simulink library "BQ76952EVM"  (R2025b)
settings: Solver=VariableStepAuto  StartTime=0.0  StopTime=10.0  RelTol=1e-3
libraries: fl_lib x55, nesl_utility x20, ee_lib x2, simulink x1
settings Model: Creator=SC-Br  LastModifiedBy=SC-Br

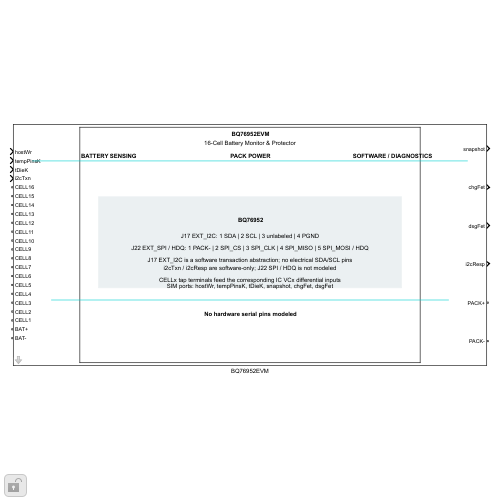
[thumbnail: Simulink's stored preview of the top-level diagram]
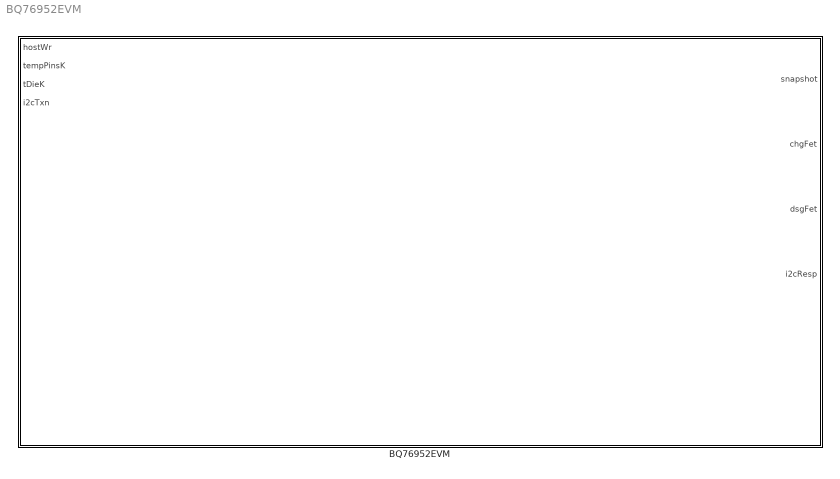
== system BQ76952EVM ==
  BQ76952EVM : Subsystem  mask(BQ76952EVM){SeriesCount=16, UsedCellMask=65535, CellSenseOhms=20, CellFilterFarads=220e-9, PositiveLinkOhms=1e-6, Preset=Generic 16S, ShuntOhms=0.001, DAConfig=6, SampleTime=0.01, PinConfig=[7 7 0 7 0 7 7 7 7], ProtEnabledA=188, ProtEnabledB=51, COV_Threshold=84, COV_Hyst=2, COV_Delay=74, CUV_Threshold=53, CUV_Hyst=2, CUV_Delay=74, OCC_Threshold=7, OCC_Delay=4, OCC_Recovery_mA=-200, OCD1_Threshold=28, OCD1_Delay=127, OCD_Recovery_mA=200, SCD_Threshold=5, SCD_Delay=2, SCD_Recovery_s=5, OTC_Threshold_C=45, OTC_Recovery_C=40, OTD_Threshold_C=60, OTD_Recovery_C=55, UTC_Threshold_C=0, UTC_Recovery_C=5, UTD_Threshold_C=-10, UTD_Recovery_C=-5, OTUT_Delay_s=2, RecoveryTime_s=3, MfgStatusInit=16, FetRon=0.001, FetGoff=1e-6, DisplayMode=Schematic View, I2CAddress=8}
      mask prompts: SeriesCount "Number of Series Cells"; UsedCellMask "Active VCell Mode (decimal)"; CellSenseOhms "VC series resistor (ohm)"; CellFilterFarads "VC filter capacitor (F)"; PositiveLinkOhms "BAT+ to PACK+ path resistance (ohm)"; Preset "Configuration preset"; ShuntOhms "Physical shunt resistance (ohm)"; DAConfig "DA_CONFIG data-memory byte"; SampleTime "Emulator sample time (s)"; PinConfig "Nine pin-configuration bytes"; ProtEnabledA "Protection enable A byte"; ProtEnabledB "Protection enable B byte"; COV_Threshold "COV threshold (50.6 mV units)"; COV_Hyst "COV recovery hysteresis (50.6 mV units)"; COV_Delay "COV delay (3.3 ms units)"; CUV_Threshold "CUV threshold (50.6 mV units)"; CUV_Hyst "CUV recovery hysteresis (50.6 mV units)"; CUV_Delay "CUV delay (3.3 ms units)"; OCC_Threshold "OCC threshold (2 mV per shunt)"; OCC_Delay "OCC delay code"; OCC_Recovery_mA "OCC recovery current (mA)"; OCD1_Threshold "OCD1 threshold (2 mV per shunt)"; OCD1_Delay "OCD1 delay code"; OCD_Recovery_mA "OCD recovery threshold (mA)"; SCD_Threshold "SCD threshold code"; SCD_Delay "SCD delay code"; SCD_Recovery_s "SCD recovery time (s)"; OTC_Threshold_C "OTC threshold (degC)"; OTC_Recovery_C "OTC recovery (degC)"; OTD_Threshold_C "OTD threshold (degC)"; OTD_Recovery_C "OTD recovery (degC)"; UTC_Threshold_C "UTC threshold (degC)"; UTC_Recovery_C "UTC recovery (degC)"; UTD_Threshold_C "UTD threshold (degC)"; UTD_Recovery_C "UTD recovery (degC)"; OTUT_Delay_s "OT/UT delay (s)"; RecoveryTime_s "Recovery time (s)"; MfgStatusInit "Manufacturing status initial word"; FetRon "Physical switch on resistance (ohm)"; FetGoff "Physical switch off conductance (S)"; DisplayMode "Display Mode"; I2CAddress "J17 I2C 7-bit address"
      mask help: Standalone behavioral BQ76952EVM. Conserving terminals retain fixed VC0-VC16 identities; use explicit external shorts for unused taps. J17 is available only through the transaction-level software interface.
      mask TypeOptions SeriesCount: 3 | 4 | 5 | 6 | 7 | 8 | 9 | 10 | 11 | 12 | 13 | 14 | 15 | 16
      mask Callback SeriesCount: n=str2double(get_param(gcb,'SeriesCount')); v=uint16(2^(n-1)-1+32768); if n==16, v=65535; end; set_param(gcb,'UsedCellMask',num2str(double(v)))
      mask TypeOptions Preset: Generic 16S | Solaris 13S | Generic 4S
      mask Callback Preset: switch get_param(gcb,'Preset'), case 'Solaris 13S', set_param(gcb,'SeriesCount','13'); set_param(gcb,'UsedCellMask','36863'); set_param(gcb,'DAConfig','6'); set_param(gcb,'ShuntOhms','0.001'); case 'Generic 4S', set_param(gcb,'SeriesCount','4'); set_param(gcb,'UsedCellMask','32775'); case 'Generic 16S', set_param(gcb,'SeriesCount','16'); set_param(gcb,'UsedCellMask','65535'); end
      mask TypeOptions DisplayMode: PCB View | Schematic View
      mask DialogControl BatteryCells Prompt: Battery / cell configuration
      mask DialogControl Current Prompt: Current sensing
      mask DialogControl Acquisition Prompt: Voltage and temperature acquisition
      mask DialogControl Protection Prompt: Protection thresholds and recovery
      mask DialogControl FETs Prompt: FET behaviour
      mask DialogControl Communications Prompt: Communications and diagnostics
      mask DialogControl ProtocolNote Prompt: J17 software transaction interface: i2cTxn (40-byte request) / i2cResp (40-byte response); supports device address, ACK/NACK, direct registers, data memory and implemented subcommands. This is not an electrical SDA/SCL waveform model. J22 SPI/HDQ is not implemented as a functional interface.
      mask Display: if DisplayMode == 1, color('white'); patch([0 1 1 0],[0 0 1 1],[1 1 1]); image(imread(fullfile(fileparts(which('BQ76952EVM')),'assets','bq76952evm_top_cropped.png')),[0.18 0.0125 0.64 0.975]); port_label('lconn',1,'CELL16'); port_label('lconn',2,'CELL15'); port_label('lconn',3,'CELL14'); port_label('lconn',4,'CELL13'); port_label('lconn',5,'CELL12'); port_label('lconn',6,'CELL11'); port_label('lconn',7,'CELL10'); port_label('lconn',8,'CELL9'); port_label('lconn',9,'CELL8'); port_label('lconn',10,'CELL7'); port_label('lconn',11,'CELL6'); port_label('lconn',12,'CELL5'); port_label('lconn',13,'CELL4'); port_label('lconn',14,'CELL3'); port_label('lconn',15,'CELL2'); port_label('lconn',16,'CELL1'); port_label('lconn',17,'BAT+'); port_label('lconn',18,'BAT-'); port_label('rconn',1,'PACK+'); port_label('rconn',2,'PACK-'); port_label('input',1,'SIM hostWr'); port_label('input',2,'SIM tempPinsK'); port_label('input',3,'SIM tDieK'); port_label('input',4,'I2C transaction request (SW)'); port_label('output',1,'SIM snapshot'); port_label('output',2,'SIM chgFet status'); port_label('output',3,'SIM dsgFet status'); port_label('output',4,'I2C transaction response (SW)'); else, color('white'); patch([0.14 0.86 0.86 0.14],[0.01 0.01 0.99 0.99],[1 1 1]); color('black'); plot([0.14 0.86 0.86 0.14 0.14],[0.01 0.01 0.99 0.99 0.01]); text(0.5,0.965,'{\bf BQ76952EVM}','horizontalAlignment','center','texmode','on'); text(0.5,0.925,'16-Cell Battery Monitor & Protector','horizontalAlignment','center'); color('black'); text(0.20,0.875,'{\bf BATTERY SENSING}','horizontalAlignment','center','texmode','on'); text(0.50,0.875,'{\bf PACK POWER}','horizontalAlignment','center','texmode','on'); text(0.80,0.875,'{\bf SOFTWARE / DIAGNOSTICS}','horizontalAlignment','center','texmode','on'); color('cyan'); plot([0.04 0.96],[0.85 0.85]); color('white'); patch([0.18 0.82 0.82 0.18],[0.32 0.32 0.70 0.70],[0.92 0.94 0.95]); color('black'); text(0.5,0.61,'{\bf BQ76952}','horizontalAlignment','center','texmode','on'); text(0.5,0.54,'J17 EXT_I2C: 1 SDA | 2 SCL | 3 unlabeled | 4 PGND','horizontalAlignment','center'); text(0.5,0.49,'J22 EXT_SPI / HDQ: 1 PACK- | 2 SPI_CS | 3 SPI_CLK | 4 SPI_MISO | 5 SPI_MOSI / HDQ','horizontalAlignment','center'); text(0.5,0.44,'J17 EXT_I2C is a software transaction abstraction; no electrical SDA/SCL pins','horizontalAlignment','center'); text(0.5,0.405,'i2cTxn / i2cResp are software-only; J22 SPI / HDQ is not modeled','horizontalAlignment','center'); text(0.5,0.355,'CELLx tap terminals feed the corresponding IC VCx differential inputs','horizontalAlignment','center'); text(0.5,0.33,'SIM ports: hostWr, tempPinsK, tDieK, snapshot, chgFet, dsgFet','horizontalAlignment','center'); color('cyan'); plot([0.08 0.92],[0.27 0.27]); color('black'); text(0.5,0.22,'{\bf No hardware serial pins modeled}','horizontalAlignment','center','texmode','on'); end

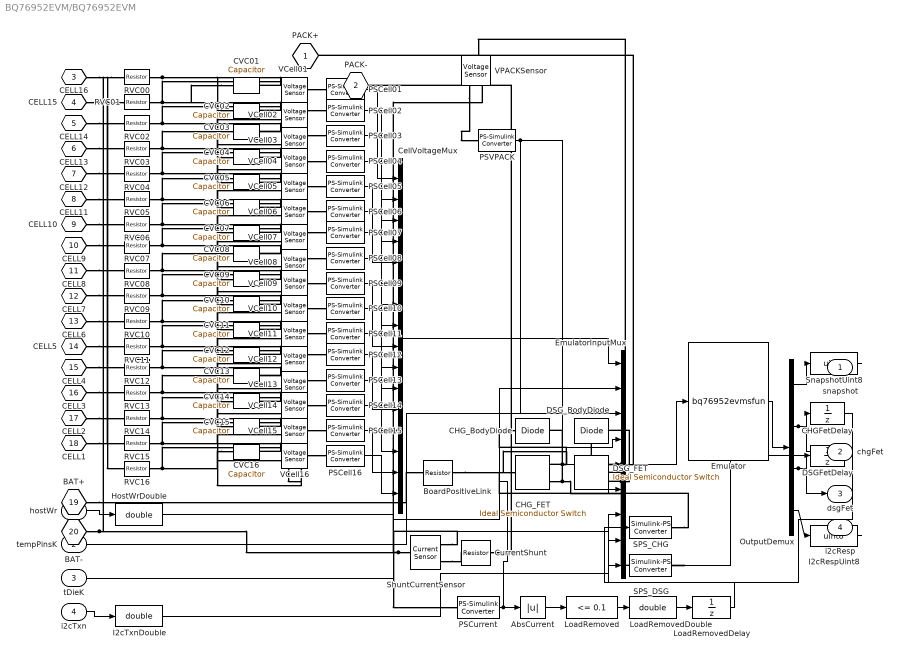
== system BQ76952EVM/BQ76952EVM ==
  hostWr : Inport  OutDataTypeStr=uint8  PortDimensions=40
  tempPinsK : Inport  Port=2  OutDataTypeStr=double  PortDimensions=9
  tDieK : Inport  Port=3  OutDataTypeStr=double  PortDimensions=1
  i2cTxn : Inport  Port=4  OutDataTypeStr=uint8  PortDimensions=40
  AbsCurrent : Abs  SaturateOnIntegerOverflow=off
  BoardPositiveLink : fl_lib/Electrical/Electrical Elements/Resistor  R=PositiveLinkOhms Ohm  i_specify=off  i_priority=None  i=0 A  i_nominal_specify=off  i_nominal_value=1  i_nominal_unit=A  v_specify=off  v_priority=None  v=0 V  v_nominal_specify=off  v_nominal_value=1  v_nominal_unit=V
  CHGFetDelay : UnitDelay  InitialCondition=1  SampleTime=SampleTime  HasFrameUpgradeWarning=on
  CHG_BodyDiode : fl_lib/Electrical/Electrical Elements/Diode  Vf=0.7 V  Ron=0.01 Ohm  Goff=FetGoff 1/Ohm  i_specify=off  i_priority=None  i=0 A  i_nominal_specify=off  i_nominal_value=1  i_nominal_unit=A  v_specify=off  v_priority=None  v=0 V  v_nominal_specify=off  v_nominal_value=1  v_nominal_unit=V
  CHG_FET : ee_lib/Semiconductors & Converters/Ideal Semiconductor Switch  port_option=ee.enum.controlport.ps  Ron=FetRon Ohm  Goff=FetGoff 1/Ohm  Vth=0.5 V  diode_param=ee.enum.semiconductors.protectionDiode.external  diode_Vf=0.8 V  diode_Ron=0.001 Ohm  diode_Goff=1e-5 1/Ohm  diode_C=50e-9 F  diode_iRM=-235 A  diode_iF=300 A  diode_idot=-50 A/us  diode_trr_param=ee.enum.converters.diodetrr.trr_factor  diode_trr_factor=3  diode_trr=15 us  diode_Qrr=1500 s*uA
  CVC01 : fl_lib/Electrical/Electrical Elements/Capacitor  c=CellFilterFarads F  r=1e-6 Ohm  g=0 1/Ohm  i_specify=off  i_priority=None  i=0 A  i_nominal_specify=off  i_nominal_value=1  i_nominal_unit=A  v_specify=off  v_priority=None  v=0 V  v_nominal_specify=off  v_nominal_value=1  v_nominal_unit=V  vc_specify=off  vc_priority=High  vc=0 V  vc_nominal_specify=off  vc_nominal_value=1  vc_nominal_unit=V
  CVC02 : fl_lib/Electrical/Electrical Elements/Capacitor  c=CellFilterFarads F  r=1e-6 Ohm  g=0 1/Ohm  i_specify=off  i_priority=None  i=0 A  i_nominal_specify=off  i_nominal_value=1  i_nominal_unit=A  v_specify=off  v_priority=None  v=0 V  v_nominal_specify=off  v_nominal_value=1  v_nominal_unit=V  vc_specify=off  vc_priority=High  vc=0 V  vc_nominal_specify=off  vc_nominal_value=1  vc_nominal_unit=V
  CVC03 : fl_lib/Electrical/Electrical Elements/Capacitor  c=CellFilterFarads F  r=1e-6 Ohm  g=0 1/Ohm  i_specify=off  i_priority=None  i=0 A  i_nominal_specify=off  i_nominal_value=1  i_nominal_unit=A  v_specify=off  v_priority=None  v=0 V  v_nominal_specify=off  v_nominal_value=1  v_nominal_unit=V  vc_specify=off  vc_priority=High  vc=0 V  vc_nominal_specify=off  vc_nominal_value=1  vc_nominal_unit=V
  CVC04 : fl_lib/Electrical/Electrical Elements/Capacitor  c=CellFilterFarads F  r=1e-6 Ohm  g=0 1/Ohm  i_specify=off  i_priority=None  i=0 A  i_nominal_specify=off  i_nominal_value=1  i_nominal_unit=A  v_specify=off  v_priority=None  v=0 V  v_nominal_specify=off  v_nominal_value=1  v_nominal_unit=V  vc_specify=off  vc_priority=High  vc=0 V  vc_nominal_specify=off  vc_nominal_value=1  vc_nominal_unit=V
  CVC05 : fl_lib/Electrical/Electrical Elements/Capacitor  c=CellFilterFarads F  r=1e-6 Ohm  g=0 1/Ohm  i_specify=off  i_priority=None  i=0 A  i_nominal_specify=off  i_nominal_value=1  i_nominal_unit=A  v_specify=off  v_priority=None  v=0 V  v_nominal_specify=off  v_nominal_value=1  v_nominal_unit=V  vc_specify=off  vc_priority=High  vc=0 V  vc_nominal_specify=off  vc_nominal_value=1  vc_nominal_unit=V
  CVC06 : fl_lib/Electrical/Electrical Elements/Capacitor  c=CellFilterFarads F  r=1e-6 Ohm  g=0 1/Ohm  i_specify=off  i_priority=None  i=0 A  i_nominal_specify=off  i_nominal_value=1  i_nominal_unit=A  v_specify=off  v_priority=None  v=0 V  v_nominal_specify=off  v_nominal_value=1  v_nominal_unit=V  vc_specify=off  vc_priority=High  vc=0 V  vc_nominal_specify=off  vc_nominal_value=1  vc_nominal_unit=V
  CVC07 : fl_lib/Electrical/Electrical Elements/Capacitor  c=CellFilterFarads F  r=1e-6 Ohm  g=0 1/Ohm  i_specify=off  i_priority=None  i=0 A  i_nominal_specify=off  i_nominal_value=1  i_nominal_unit=A  v_specify=off  v_priority=None  v=0 V  v_nominal_specify=off  v_nominal_value=1  v_nominal_unit=V  vc_specify=off  vc_priority=High  vc=0 V  vc_nominal_specify=off  vc_nominal_value=1  vc_nominal_unit=V
  CVC08 : fl_lib/Electrical/Electrical Elements/Capacitor  c=CellFilterFarads F  r=1e-6 Ohm  g=0 1/Ohm  i_specify=off  i_priority=None  i=0 A  i_nominal_specify=off  i_nominal_value=1  i_nominal_unit=A  v_specify=off  v_priority=None  v=0 V  v_nominal_specify=off  v_nominal_value=1  v_nominal_unit=V  vc_specify=off  vc_priority=High  vc=0 V  vc_nominal_specify=off  vc_nominal_value=1  vc_nominal_unit=V
  CVC09 : fl_lib/Electrical/Electrical Elements/Capacitor  c=CellFilterFarads F  r=1e-6 Ohm  g=0 1/Ohm  i_specify=off  i_priority=None  i=0 A  i_nominal_specify=off  i_nominal_value=1  i_nominal_unit=A  v_specify=off  v_priority=None  v=0 V  v_nominal_specify=off  v_nominal_value=1  v_nominal_unit=V  vc_specify=off  vc_priority=High  vc=0 V  vc_nominal_specify=off  vc_nominal_value=1  vc_nominal_unit=V
  CVC{10..16} (7 alike) : fl_lib/Electrical/Electrical Elements/Capacitor  c=CellFilterFarads F  r=1e-6 Ohm  g=0 1/Ohm  i_specify=off  i_priority=None  i=0 A  i_nominal_specify=off  i_nominal_value=1  i_nominal_unit=A  v_specify=off  v_priority=None  v=0 V  v_nominal_specify=off  v_nominal_value=1  v_nominal_unit=V  vc_specify=off  vc_priority=High  vc=0 V  vc_nominal_specify=off  vc_nominal_value=1  vc_nominal_unit=V
  CellVoltageMux : Mux  Inputs=16
  CurrentShunt : fl_lib/Electrical/Electrical Elements/Resistor  R=ShuntOhms Ohm  i_specify=off  i_priority=None  i=0 A  i_nominal_specify=off  i_nominal_value=1  i_nominal_unit=A  v_specify=off  v_priority=None  v=0 V  v_nominal_specify=off  v_nominal_value=1  v_nominal_unit=V
  DSGFetDelay : UnitDelay  InitialCondition=1  SampleTime=SampleTime  HasFrameUpgradeWarning=on
  DSG_BodyDiode : fl_lib/Electrical/Electrical Elements/Diode  Vf=0.7 V  Ron=0.01 Ohm  Goff=FetGoff 1/Ohm  i_specify=off  i_priority=None  i=0 A  i_nominal_specify=off  i_nominal_value=1  i_nominal_unit=A  v_specify=off  v_priority=None  v=0 V  v_nominal_specify=off  v_nominal_value=1  v_nominal_unit=V
  DSG_FET : ee_lib/Semiconductors & Converters/Ideal Semiconductor Switch  port_option=ee.enum.controlport.ps  Ron=FetRon Ohm  Goff=FetGoff 1/Ohm  Vth=0.5 V  diode_param=ee.enum.semiconductors.protectionDiode.external  diode_Vf=0.8 V  diode_Ron=0.001 Ohm  diode_Goff=1e-5 1/Ohm  diode_C=50e-9 F  diode_iRM=-235 A  diode_iF=300 A  diode_idot=-50 A/us  diode_trr_param=ee.enum.converters.diodetrr.trr_factor  diode_trr_factor=3  diode_trr=15 us  diode_Qrr=1500 s*uA
  Emulator : S-Function  FunctionName=bq76952evmsfun  Parameters=[SampleTime; UsedCellMask; round(ShuntOhms*1e6); DAConfig; ProtEnabledA; ProtEnabledB; MfgStatusInit; COV_Threshold; COV_Hyst; COV_Delay; CUV_Threshold; CUV_Hyst; CUV_Delay; OCC_Threshold; OCC_Delay; OCC_Recovery_mA; OCD1_Threshold; OCD1_Delay; OCD_Recovery_mA; SCD_Threshold; SCD_Delay; SCD_Recovery_s; OTC_Threshold_C; OTC_Recovery_C; OTD_Threshold_C; OTD_Recovery_C; UTC_Threshold_C; UTC_Recovery_C; UTD_Threshold_C; UTD_Recovery_C; OTUT_Delay_s; RecoveryTime_s; PinConfig(:); I2CAddress]  SFunctionDeploymentMode=off  EnableBusSupport=off
  EmulatorInputMux : Mux  Inputs=9
  HostWrDouble : DataTypeConversion  OutDataTypeStr=double  SaturateOnIntegerOverflow=off  RndMeth=Floor
  I2cRespUint8 : DataTypeConversion  OutDataTypeStr=uint8  SaturateOnIntegerOverflow=off  RndMeth=Floor
  I2cTxnDouble : DataTypeConversion  OutDataTypeStr=double  SaturateOnIntegerOverflow=off  RndMeth=Floor
  LoadRemoved : simulink/Logic and Bit Operations/Compare To Constant  relop=<=  const=0.1  OutDataTypeStr=boolean
  LoadRemovedDelay : UnitDelay  SampleTime=SampleTime  HasFrameUpgradeWarning=on
  LoadRemovedDouble : DataTypeConversion  OutDataTypeStr=double  SaturateOnIntegerOverflow=off  RndMeth=Floor
  OutputDemux : Demux  Outputs=[144 1 1 40]
  PSCell01 : nesl_utility/PS-Simulink Converter  PhysicalDomain=network_engine_domain  SubClassName=ps_output  LeftPortType=input  RightPortType=output  PseudoPeriodic=off  Frequencies=[]  VectorFormat=inherit  Unit=inherit  AffineConversion=off
  PSCell02 : nesl_utility/PS-Simulink Converter  PhysicalDomain=network_engine_domain  SubClassName=ps_output  LeftPortType=input  RightPortType=output  PseudoPeriodic=off  Frequencies=[]  VectorFormat=inherit  Unit=inherit  AffineConversion=off
  PSCell03 : nesl_utility/PS-Simulink Converter  PhysicalDomain=network_engine_domain  SubClassName=ps_output  LeftPortType=input  RightPortType=output  PseudoPeriodic=off  Frequencies=[]  VectorFormat=inherit  Unit=inherit  AffineConversion=off
  PSCell04 : nesl_utility/PS-Simulink Converter  PhysicalDomain=network_engine_domain  SubClassName=ps_output  LeftPortType=input  RightPortType=output  PseudoPeriodic=off  Frequencies=[]  VectorFormat=inherit  Unit=inherit  AffineConversion=off
  PSCell05 : nesl_utility/PS-Simulink Converter  PhysicalDomain=network_engine_domain  SubClassName=ps_output  LeftPortType=input  RightPortType=output  PseudoPeriodic=off  Frequencies=[]  VectorFormat=inherit  Unit=inherit  AffineConversion=off
  PSCell06 : nesl_utility/PS-Simulink Converter  PhysicalDomain=network_engine_domain  SubClassName=ps_output  LeftPortType=input  RightPortType=output  PseudoPeriodic=off  Frequencies=[]  VectorFormat=inherit  Unit=inherit  AffineConversion=off
  PSCell07 : nesl_utility/PS-Simulink Converter  PhysicalDomain=network_engine_domain  SubClassName=ps_output  LeftPortType=input  RightPortType=output  PseudoPeriodic=off  Frequencies=[]  VectorFormat=inherit  Unit=inherit  AffineConversion=off
  PSCell08 : nesl_utility/PS-Simulink Converter  PhysicalDomain=network_engine_domain  SubClassName=ps_output  LeftPortType=input  RightPortType=output  PseudoPeriodic=off  Frequencies=[]  VectorFormat=inherit  Unit=inherit  AffineConversion=off
  PSCell09 : nesl_utility/PS-Simulink Converter  PhysicalDomain=network_engine_domain  SubClassName=ps_output  LeftPortType=input  RightPortType=output  PseudoPeriodic=off  Frequencies=[]  VectorFormat=inherit  Unit=inherit  AffineConversion=off
  PSCell{10..16} (7 alike) : nesl_utility/PS-Simulink Converter  PhysicalDomain=network_engine_domain  SubClassName=ps_output  LeftPortType=input  RightPortType=output  PseudoPeriodic=off  Frequencies=[]  VectorFormat=inherit  Unit=inherit  AffineConversion=off
  PSCurrent : nesl_utility/PS-Simulink Converter  PhysicalDomain=network_engine_domain  SubClassName=ps_output  LeftPortType=input  RightPortType=output  PseudoPeriodic=off  Frequencies=[]  VectorFormat=inherit  Unit=inherit  AffineConversion=off
  PSVPACK : nesl_utility/PS-Simulink Converter  PhysicalDomain=network_engine_domain  SubClassName=ps_output  LeftPortType=input  RightPortType=output  PseudoPeriodic=off  Frequencies=[]  VectorFormat=inherit  Unit=inherit  AffineConversion=off
  RVC00 : fl_lib/Electrical/Electrical Elements/Resistor  R=CellSenseOhms Ohm  i_specify=off  i_priority=None  i=0 A  i_nominal_specify=off  i_nominal_value=1  i_nominal_unit=A  v_specify=off  v_priority=None  v=0 V  v_nominal_specify=off  v_nominal_value=1  v_nominal_unit=V
  RVC01 : fl_lib/Electrical/Electrical Elements/Resistor  R=CellSenseOhms Ohm  i_specify=off  i_priority=None  i=0 A  i_nominal_specify=off  i_nominal_value=1  i_nominal_unit=A  v_specify=off  v_priority=None  v=0 V  v_nominal_specify=off  v_nominal_value=1  v_nominal_unit=V
  RVC02 : fl_lib/Electrical/Electrical Elements/Resistor  R=CellSenseOhms Ohm  i_specify=off  i_priority=None  i=0 A  i_nominal_specify=off  i_nominal_value=1  i_nominal_unit=A  v_specify=off  v_priority=None  v=0 V  v_nominal_specify=off  v_nominal_value=1  v_nominal_unit=V
  RVC03 : fl_lib/Electrical/Electrical Elements/Resistor  R=CellSenseOhms Ohm  i_specify=off  i_priority=None  i=0 A  i_nominal_specify=off  i_nominal_value=1  i_nominal_unit=A  v_specify=off  v_priority=None  v=0 V  v_nominal_specify=off  v_nominal_value=1  v_nominal_unit=V
  RVC04 : fl_lib/Electrical/Electrical Elements/Resistor  R=CellSenseOhms Ohm  i_specify=off  i_priority=None  i=0 A  i_nominal_specify=off  i_nominal_value=1  i_nominal_unit=A  v_specify=off  v_priority=None  v=0 V  v_nominal_specify=off  v_nominal_value=1  v_nominal_unit=V
  RVC05 : fl_lib/Electrical/Electrical Elements/Resistor  R=CellSenseOhms Ohm  i_specify=off  i_priority=None  i=0 A  i_nominal_specify=off  i_nominal_value=1  i_nominal_unit=A  v_specify=off  v_priority=None  v=0 V  v_nominal_specify=off  v_nominal_value=1  v_nominal_unit=V
  RVC06 : fl_lib/Electrical/Electrical Elements/Resistor  R=CellSenseOhms Ohm  i_specify=off  i_priority=None  i=0 A  i_nominal_specify=off  i_nominal_value=1  i_nominal_unit=A  v_specify=off  v_priority=None  v=0 V  v_nominal_specify=off  v_nominal_value=1  v_nominal_unit=V
  RVC07 : fl_lib/Electrical/Electrical Elements/Resistor  R=CellSenseOhms Ohm  i_specify=off  i_priority=None  i=0 A  i_nominal_specify=off  i_nominal_value=1  i_nominal_unit=A  v_specify=off  v_priority=None  v=0 V  v_nominal_specify=off  v_nominal_value=1  v_nominal_unit=V
  RVC08 : fl_lib/Electrical/Electrical Elements/Resistor  R=CellSenseOhms Ohm  i_specify=off  i_priority=None  i=0 A  i_nominal_specify=off  i_nominal_value=1  i_nominal_unit=A  v_specify=off  v_priority=None  v=0 V  v_nominal_specify=off  v_nominal_value=1  v_nominal_unit=V
  RVC09 : fl_lib/Electrical/Electrical Elements/Resistor  R=CellSenseOhms Ohm  i_specify=off  i_priority=None  i=0 A  i_nominal_specify=off  i_nominal_value=1  i_nominal_unit=A  v_specify=off  v_priority=None  v=0 V  v_nominal_specify=off  v_nominal_value=1  v_nominal_unit=V
  RVC{10..16} (7 alike) : fl_lib/Electrical/Electrical Elements/Resistor  R=CellSenseOhms Ohm  i_specify=off  i_priority=None  i=0 A  i_nominal_specify=off  i_nominal_value=1  i_nominal_unit=A  v_specify=off  v_priority=None  v=0 V  v_nominal_specify=off  v_nominal_value=1  v_nominal_unit=V
  SPS_CHG : nesl_utility/Simulink-PS Converter  PhysicalDomain=network_engine_domain  SubClassName=ps_input  LeftPortType=input  RightPortType=output  PseudoPeriodic=off  Frequencies=[]  NoiseDistribution=none  NoiseParameters=[]  Unit=1  AffineConversion=off  FilteringAndDerivatives=provide  SimscapeFilterOrder=1  InputFilterTimeConstant=0.001  UdotUserProvided=0
  SPS_DSG : nesl_utility/Simulink-PS Converter  PhysicalDomain=network_engine_domain  SubClassName=ps_input  LeftPortType=input  RightPortType=output  PseudoPeriodic=off  Frequencies=[]  NoiseDistribution=none  NoiseParameters=[]  Unit=1  AffineConversion=off  FilteringAndDerivatives=provide  SimscapeFilterOrder=1  InputFilterTimeConstant=0.001  UdotUserProvided=0
  ShuntCurrentSensor : fl_lib/Electrical/Electrical Sensors/Current Sensor
  SnapshotUint8 : DataTypeConversion  OutDataTypeStr=uint8  SaturateOnIntegerOverflow=off  RndMeth=Floor
  VCell01 : fl_lib/Electrical/Electrical Sensors/Voltage Sensor
  VCell02 : fl_lib/Electrical/Electrical Sensors/Voltage Sensor
  VCell03 : fl_lib/Electrical/Electrical Sensors/Voltage Sensor
  VCell04 : fl_lib/Electrical/Electrical Sensors/Voltage Sensor
  VCell05 : fl_lib/Electrical/Electrical Sensors/Voltage Sensor
  VCell06 : fl_lib/Electrical/Electrical Sensors/Voltage Sensor
  VCell07 : fl_lib/Electrical/Electrical Sensors/Voltage Sensor
  VCell08 : fl_lib/Electrical/Electrical Sensors/Voltage Sensor
  VCell09 : fl_lib/Electrical/Electrical Sensors/Voltage Sensor
  VCell{10..16} (7 alike) : fl_lib/Electrical/Electrical Sensors/Voltage Sensor
  VPACKSensor : fl_lib/Electrical/Electrical Sensors/Voltage Sensor
  PACK+ : PMIOPort  Side=Right
  PACK- : PMIOPort  Port=2  Side=Right
  CELL16 : PMIOPort  Port=3  Side=Left
  CELL15 : PMIOPort  Port=4  Side=Left
  CELL14 : PMIOPort  Port=5  Side=Left
  CELL13 : PMIOPort  Port=6  Side=Left
  CELL12 : PMIOPort  Port=7  Side=Left
  CELL11 : PMIOPort  Port=8  Side=Left
  CELL10 : PMIOPort  Port=9  Side=Left
  CELL9 : PMIOPort  Port=10  Side=Left
  CELL8 : PMIOPort  Port=11  Side=Left
  CELL7 : PMIOPort  Port=12  Side=Left
  CELL6 : PMIOPort  Port=13  Side=Left
  CELL5 : PMIOPort  Port=14  Side=Left
  CELL4 : PMIOPort  Port=15  Side=Left
  CELL3 : PMIOPort  Port=16  Side=Left
  CELL2 : PMIOPort  Port=17  Side=Left
  CELL1 : PMIOPort  Port=18  Side=Left
  BAT+ : PMIOPort  Port=19  Side=Left
  BAT- : PMIOPort  Port=20  Side=Left
  snapshot : Outport  OutDataTypeStr=uint8  PortDimensions=144
  chgFet : Outport  Port=2  OutDataTypeStr=double  PortDimensions=1
  dsgFet : Outport  Port=3  OutDataTypeStr=double  PortDimensions=1
  i2cResp : Outport  Port=4  OutDataTypeStr=uint8  PortDimensions=40
  wires:
  PSCell01/1 -> CellVoltageMux/1
  PSCell02/1 -> CellVoltageMux/2
  PSCell03/1 -> CellVoltageMux/3
  PSCell04/1 -> CellVoltageMux/4
  PSCell05/1 -> CellVoltageMux/5
  PSCell06/1 -> CellVoltageMux/6
  PSCell07/1 -> CellVoltageMux/7
  PSCell08/1 -> CellVoltageMux/8
  PSCell09/1 -> CellVoltageMux/9
  PSCell10/1 -> CellVoltageMux/10
  PSCell11/1 -> CellVoltageMux/11
  PSCell12/1 -> CellVoltageMux/12
  PSCell13/1 -> CellVoltageMux/13
  PSCell14/1 -> CellVoltageMux/14
  PSCell15/1 -> CellVoltageMux/15
  PSCell16/1 -> CellVoltageMux/16
  CellVoltageMux/1 -> EmulatorInputMux/1
  PSCurrent/1 -> AbsCurrent/1, EmulatorInputMux/2
  AbsCurrent/1 -> LoadRemoved/1
  LoadRemoved/1 -> LoadRemovedDouble/1
  LoadRemovedDouble/1 -> LoadRemovedDelay/1
  tempPinsK/1 -> EmulatorInputMux/3
  tDieK/1 -> EmulatorInputMux/4
  PSVPACK/1 -> EmulatorInputMux/5, EmulatorInputMux/6
  LoadRemovedDelay/1 -> EmulatorInputMux/7
  hostWr/1 -> HostWrDouble/1
  HostWrDouble/1 -> EmulatorInputMux/8
  i2cTxn/1 -> I2cTxnDouble/1
  I2cTxnDouble/1 -> EmulatorInputMux/9
  EmulatorInputMux/1 -> Emulator/1
  Emulator/1 -> OutputDemux/1
  OutputDemux/1 -> SnapshotUint8/1
  OutputDemux/2 -> CHGFetDelay/1, chgFet/1
  OutputDemux/3 -> DSGFetDelay/1, dsgFet/1
  CHGFetDelay/1 -> SPS_CHG/1
  DSGFetDelay/1 -> SPS_DSG/1
  SnapshotUint8/1 -> snapshot/1
  OutputDemux/4 -> I2cRespUint8/1
  I2cRespUint8/1 -> i2cResp/1
  connections:
  RVC00/LConn1 -- BAT-/RConn1 -- ShuntCurrentSensor/LConn1 -- VPACKSensor/RConn2
  CELL1/RConn1 -- RVC01/LConn1
  CELL2/RConn1 -- RVC02/LConn1
  CELL3/RConn1 -- RVC03/LConn1
  CELL4/RConn1 -- RVC04/LConn1
  CELL5/RConn1 -- RVC05/LConn1
  CELL6/RConn1 -- RVC06/LConn1
  CELL7/RConn1 -- RVC07/LConn1
  CELL8/RConn1 -- RVC08/LConn1
  CELL9/RConn1 -- RVC09/LConn1
  CELL10/RConn1 -- RVC10/LConn1
  CELL11/RConn1 -- RVC11/LConn1
  CELL12/RConn1 -- RVC12/LConn1
  CELL13/RConn1 -- RVC13/LConn1
  CELL14/RConn1 -- RVC14/LConn1
  CELL15/RConn1 -- RVC15/LConn1
  CELL16/RConn1 -- RVC16/LConn1
  CVC01/LConn1 -- RVC01/RConn1 -- VCell01/LConn1 -- CVC02/RConn1 -- VCell02/RConn2
  CVC01/RConn1 -- RVC00/RConn1 -- VCell01/RConn2
  VCell01/RConn1 -- PSCell01/LConn1
  CVC02/LConn1 -- RVC02/RConn1 -- VCell02/LConn1 -- CVC03/RConn1 -- VCell03/RConn2
  VCell02/RConn1 -- PSCell02/LConn1
  CVC03/LConn1 -- RVC03/RConn1 -- VCell03/LConn1 -- CVC04/RConn1 -- VCell04/RConn2
  VCell03/RConn1 -- PSCell03/LConn1
  CVC04/LConn1 -- RVC04/RConn1 -- VCell04/LConn1 -- CVC05/RConn1 -- VCell05/RConn2
  VCell04/RConn1 -- PSCell04/LConn1
  CVC05/LConn1 -- RVC05/RConn1 -- VCell05/LConn1 -- CVC06/RConn1 -- VCell06/RConn2
  VCell05/RConn1 -- PSCell05/LConn1
  CVC06/LConn1 -- RVC06/RConn1 -- VCell06/LConn1 -- CVC07/RConn1 -- VCell07/RConn2
  VCell06/RConn1 -- PSCell06/LConn1
  CVC07/LConn1 -- RVC07/RConn1 -- VCell07/LConn1 -- CVC08/RConn1 -- VCell08/RConn2
  VCell07/RConn1 -- PSCell07/LConn1
  CVC08/LConn1 -- RVC08/RConn1 -- VCell08/LConn1 -- CVC09/RConn1 -- VCell09/RConn2
  VCell08/RConn1 -- PSCell08/LConn1
  CVC09/LConn1 -- RVC09/RConn1 -- VCell09/LConn1 -- CVC10/RConn1 -- VCell10/RConn2
  VCell09/RConn1 -- PSCell09/LConn1
  CVC10/LConn1 -- RVC10/RConn1 -- VCell10/LConn1 -- CVC11/RConn1 -- VCell11/RConn2
  VCell10/RConn1 -- PSCell10/LConn1
  CVC11/LConn1 -- RVC11/RConn1 -- VCell11/LConn1 -- CVC12/RConn1 -- VCell12/RConn2
  VCell11/RConn1 -- PSCell11/LConn1
  CVC12/LConn1 -- RVC12/RConn1 -- VCell12/LConn1 -- CVC13/RConn1 -- VCell13/RConn2
  VCell12/RConn1 -- PSCell12/LConn1
  CVC13/LConn1 -- RVC13/RConn1 -- VCell13/LConn1 -- CVC14/RConn1 -- VCell14/RConn2
  VCell13/RConn1 -- PSCell13/LConn1
  CVC14/LConn1 -- RVC14/RConn1 -- VCell14/LConn1 -- CVC15/RConn1 -- VCell15/RConn2
  VCell14/RConn1 -- PSCell14/LConn1
  CVC15/LConn1 -- RVC15/RConn1 -- VCell15/LConn1 -- CVC16/RConn1 -- VCell16/RConn2
  VCell15/RConn1 -- PSCell15/LConn1
  CVC16/LConn1 -- RVC16/RConn1 -- VCell16/LConn1
  VCell16/RConn1 -- PSCell16/LConn1
  ShuntCurrentSensor/RConn2 -- CurrentShunt/LConn1
  CurrentShunt/RConn1 -- PACK-/RConn1
  BAT+/RConn1 -- BoardPositiveLink/LConn1
  CHG_FET/RConn1 -- BoardPositiveLink/RConn1 -- CHG_BodyDiode/LConn1
  CHG_FET/RConn2 -- CHG_BodyDiode/RConn1 -- DSG_FET/RConn2 -- DSG_BodyDiode/RConn1
  PACK+/RConn1 -- DSG_FET/RConn1 -- DSG_BodyDiode/LConn1 -- VPACKSensor/LConn1
  VPACKSensor/RConn1 -- PSVPACK/LConn1
  SPS_CHG/RConn1 -- CHG_FET/LConn1
  SPS_DSG/RConn1 -- DSG_FET/LConn1
  ShuntCurrentSensor/RConn1 -- PSCurrent/LConn1
